simulink model "Boost_LQR_lim"  (R2026b)
settings: Solver=FixedStepDiscrete  StopTime=Tfin  FixedStep=Ts
InitFcn:
  | init_BOOT
values from neighbouring files (symbols this model uses):
  t1 = 0.025    [init_BOOT.m]
  t2 = 1    [init_BOOT.m]
  t3 = 2    [init_BOOT.m]
  Ts = evalin('base', 'Ts')    [ejecutar_PIL.m]    (also in init_BOOT.m = 0.00025; prueba_independencia_PIL.m)
  Vref_1 = 12    [init_BOOT.m]
  Vref_2 = 12    [init_BOOT.m]
  Vref_3 = 12    [init_BOOT.m]
undefined symbols (not defined in the file or in its folder): den_Gp_d, dspblkCoreblockFVToolHelper, gcbh, num_Gp_d
settings Model: Creator=Usuario  LastModifiedBy=matia
settings DataIOCC: ReturnWorkspaceOutputs=off
settings RTWCC: CodeExecutionProfiling=on

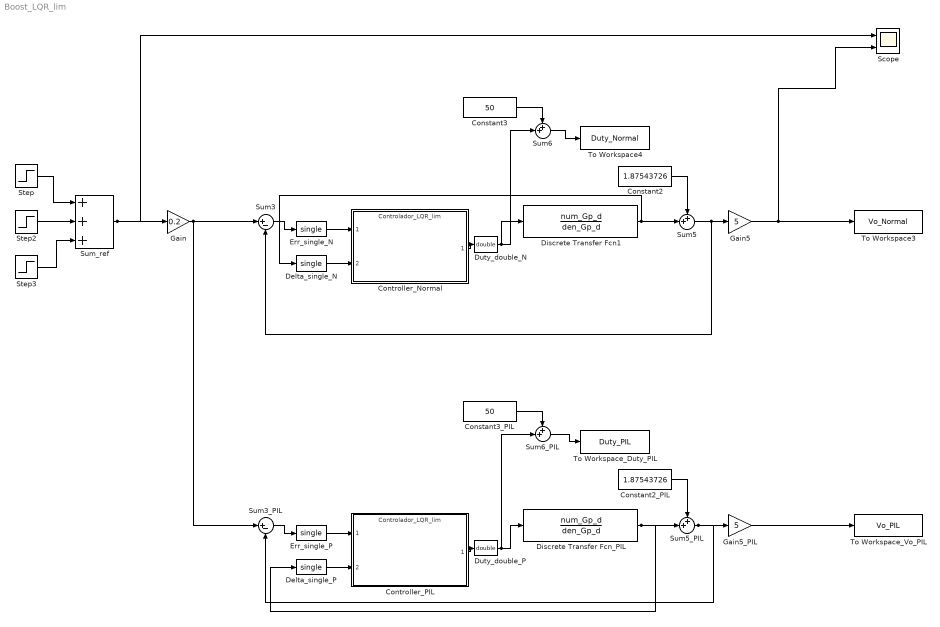
== system Boost_LQR_lim ==
  Constant2 : Constant  Value=1.87543726
  Constant2_PIL : Constant  Value=1.87543726
  Constant3 : Constant  Value=50
  Constant3_PIL : Constant  Value=50
  Controller_Normal : ModelReference  ModelNameDialog=Controlador_LQR_lim  SimulationMode=Normal  ModelReferenceVersion=2.2
  Controller_PIL : ModelReference  ModelNameDialog=Controlador_LQR_lim  SimulationMode=Processor-in-the-loop (PIL)  ModelReferenceVersion=2.2
  Delta_single_N : DataTypeConversion  OutDataTypeStr=single  SaturateOnIntegerOverflow=off  RndMeth=Floor
  Delta_single_P : DataTypeConversion  OutDataTypeStr=single  SaturateOnIntegerOverflow=off  RndMeth=Floor
  Discrete Transfer Fcn1 : DiscreteTransferFcn  LoadFcn=dspblkCoreblockFVToolHelper(gcbh,'load');  Numerator=num_Gp_d  Denominator=den_Gp_d
      settings: CopyFcn=dspblkCoreblockFVToolHelper(gcbh,'copy');  DeleteFcn=dspblkCoreblockFVToolHelper(gcbh,'close');  ModelCloseFcn=dspblkCoreblockFVToolHelper(gcbh,'close');  PreSaveFcn=dspblkCoreblockFVToolHelper(gcbh,'presave');  PostSaveFcn=dspblkCoreblockFVToolHelper(gcbh,'postsave');  CloseFcn=dspblkCoreblockFVToolHelper(gcbh,'close');
  Discrete Transfer Fcn_PIL : DiscreteTransferFcn  LoadFcn=dspblkCoreblockFVToolHelper(gcbh,'load');  Numerator=num_Gp_d  Denominator=den_Gp_d
      settings: CopyFcn=dspblkCoreblockFVToolHelper(gcbh,'copy');  DeleteFcn=dspblkCoreblockFVToolHelper(gcbh,'close');  ModelCloseFcn=dspblkCoreblockFVToolHelper(gcbh,'close');  PreSaveFcn=dspblkCoreblockFVToolHelper(gcbh,'presave');  PostSaveFcn=dspblkCoreblockFVToolHelper(gcbh,'postsave');  CloseFcn=dspblkCoreblockFVToolHelper(gcbh,'close');
  Duty_double_N : DataTypeConversion  OutDataTypeStr=double  SaturateOnIntegerOverflow=off  RndMeth=Floor
  Duty_double_P : DataTypeConversion  OutDataTypeStr=double  SaturateOnIntegerOverflow=off  RndMeth=Floor
  Err_single_N : DataTypeConversion  OutDataTypeStr=single  SaturateOnIntegerOverflow=off  RndMeth=Floor
  Err_single_P : DataTypeConversion  OutDataTypeStr=single  SaturateOnIntegerOverflow=off  RndMeth=Floor
  Gain : Gain  Gain=0.2
  Gain5 : Gain  Gain=5
  Gain5_PIL : Gain  Gain=5
  Scope : Scope  NumInputPorts=2
      settings: ActiveDisplayYMinimum=9.04733262947689  ActiveDisplayYMaximum=12.345869334708013
  Step : Step  Time=t1  InitialValue=Vref_0  FinalValue=Vref_1  SampleTime=Ts
  Step2 : Step  Time=t2  FinalValue=Vref_2-Vref_1  SampleTime=Ts
  Step3 : Step  Time=t3  FinalValue=Vref_3-Vref_2  SampleTime=Ts
  Sum3 : Sum  Inputs=|+-
  Sum3_PIL : Sum  Inputs=|+-
  Sum5 : Sum  Inputs=++|
  Sum5_PIL : Sum  Inputs=++|
  Sum6 : Sum  Inputs=++|
  Sum6_PIL : Sum  Inputs=++|
  Sum_ref : Sum  Inputs=+++
  To Workspace3 : ToWorkspace  VariableName=Vo_Normal  SaveFormat=Timeseries  SampleTime=Ts
  To Workspace4 : ToWorkspace  VariableName=Duty_Normal  SaveFormat=Timeseries  SampleTime=Ts
  To Workspace_Duty_PIL : ToWorkspace  VariableName=Duty_PIL  SaveFormat=Timeseries  SampleTime=Ts
  To Workspace_Vo_PIL : ToWorkspace  VariableName=Vo_PIL  SaveFormat=Timeseries  SampleTime=Ts
  wires:
  Gain/1 -> Sum3/1, Sum3_PIL/1
  Discrete Transfer Fcn1/1 -> Sum5/2, Delta_single_N/1
  Constant2/1 -> Sum5/1
  Sum5/1 -> Sum3/2, Gain5/1
  Constant3/1 -> Sum6/1
  Sum6/1 -> To Workspace4/1
  Gain5/1 -> Scope/2, To Workspace3/1
  Sum3/1 -> Err_single_N/1
  Err_single_N/1 -> Controller_Normal/1
  Delta_single_N/1 -> Controller_Normal/2
  Controller_Normal/1 -> Duty_double_N/1
  Duty_double_N/1 -> Sum6/2, Discrete Transfer Fcn1/1
  Sum3_PIL/1 -> Err_single_P/1
  Err_single_P/1 -> Controller_PIL/1
  Discrete Transfer Fcn_PIL/1 -> Delta_single_P/1, Sum5_PIL/2
  Delta_single_P/1 -> Controller_PIL/2
  Controller_PIL/1 -> Duty_double_P/1
  Duty_double_P/1 -> Discrete Transfer Fcn_PIL/1, Sum6_PIL/2
  Constant3_PIL/1 -> Sum6_PIL/1
  Sum6_PIL/1 -> To Workspace_Duty_PIL/1
  Constant2_PIL/1 -> Sum5_PIL/1
  Sum5_PIL/1 -> Sum3_PIL/2, Gain5_PIL/1
  Gain5_PIL/1 -> To Workspace_Vo_PIL/1
  Step/1 -> Sum_ref/1
  Step2/1 -> Sum_ref/2
  Step3/1 -> Sum_ref/3
  Sum_ref/1 -> Scope/1, Gain/1
